simulink model "WBR_control"  (R2021b)
settings: Solver=ode4  StartTime=0.0  StopTime=12  FixedStep=1e-4  RelTol=1e-3
undefined symbols (not defined in the file): leg_controller, leg_l1, leg_l2, leg_model, leg_r1, leg_r2, locomotion_controller, param, sigbuilder_block, wheel_l, wheel_r, X, Y, Z
libraries: sm_lib x110, nesl_utility x29, slpidlib x2
(part 4 of 4)

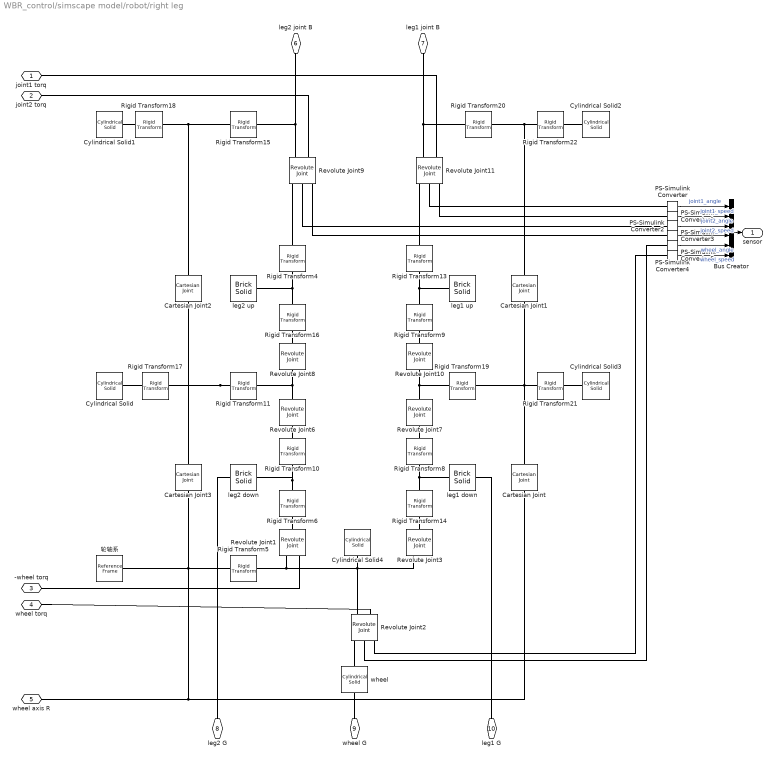
== system WBR_control/simscape model/robot/right leg ==
  Bus Creator : BusCreator  Inputs=6
  Cartesian Joint{,1..3} (4 alike) : sm_lib/Joints/Cartesian Joint  JointMode=Normal  SenseConstraintForce=off  SenseConstraintForceX=off  SenseConstraintForceY=off  SenseConstraintForceZ=off  SenseConstraintTorque=off  SenseConstraintTorqueX=off  SenseConstraintTorqueY=off  SenseConstraintTorqueZ=off  SenseTotalForce=off  SenseTotalForceX=off  SenseTotalForceY=off  SenseTotalForceZ=off  SenseTotalTorque=off  SenseTotalTorqueX=off  SenseTotalTorqueY=off  SenseTotalTorqueZ=off  CompositeWrenchDir=FollowerOnBase  CompositeWrenchFrame=BaseFrame  PxEquilibriumPosition=0  PxEquilibriumPositionUnits=m  PxSpringStiffness=0  PxSpringStiffnessUnits=N/m  PxDampingCoefficient=0  PxDampingCoefficientUnits=N/(m/s)  PxTorqueActuationMode=NoTorque  PxMotionActuationMode=ComputedMotion  PxSensePosition=off  PxSenseVelocity=off  PxSenseAcceleration=off  PxSenseTorqueForce=off  PxSenseLowerLimitTorqueForce=off  PxSenseUpperLimitTorqueForce=off  PxLowerLimitSpecify=off  PxLowerLimitBound=-1  PxLowerLimitBoundUnits=m  PxLowerLimitStiffness=1e6  PxLowerLimitStiffnessUnits=N/m  PxLowerLimitDamping=1e3  PxLowerLimitDampingUnits=N/(m/s)  PxLowerLimitTransitionRegionWidth=1e-4  PxLowerLimitTransitionRegionWidthUnits=m  PxUpperLimitSpecify=off  PxUpperLimitBound=1  PxUpperLimitBoundUnits=m  PxUpperLimitStiffness=1e6  PxUpperLimitStiffnessUnits=N/m  PxUpperLimitDamping=1e3  PxUpperLimitDampingUnits=N/(m/s)  PxUpperLimitTransitionRegionWidth=1e-4  PxUpperLimitTransitionRegionWidthUnits=m  PxPositionTargetSpecify=off  PxPositionTargetPriority=High  PxPositionTargetValue=0  PxPositionTargetValueUnits=m  PxVelocityTargetSpecify=off  PxVelocityTargetPriority=High  PxVelocityTargetValue=0  PxVelocityTargetValueUnits=m/s  PyEquilibriumPosition=0  PyEquilibriumPositionUnits=m  PySpringStiffness=0  PySpringStiffnessUnits=N/m  PyDampingCoefficient=0  PyDampingCoefficientUnits=N/(m/s)  PyTorqueActuationMode=NoTorque  PyMotionActuationMode=ComputedMotion  PySensePosition=off  PySenseVelocity=off  PySenseAcceleration=off  PySenseTorqueForce=off  PySenseLowerLimitTorqueForce=off  PySenseUpperLimitTorqueForce=off  PyLowerLimitSpecify=off  PyLowerLimitBound=-1  PyLowerLimitBoundUnits=m  PyLowerLimitStiffness=1e6  PyLowerLimitStiffnessUnits=N/m  PyLowerLimitDamping=1e3  PyLowerLimitDampingUnits=N/(m/s)  PyLowerLimitTransitionRegionWidth=1e-4  PyLowerLimitTransitionRegionWidthUnits=m  PyUpperLimitSpecify=off  PyUpperLimitBound=1  PyUpperLimitBoundUnits=m  PyUpperLimitStiffness=1e6  PyUpperLimitStiffnessUnits=N/m  PyUpperLimitDamping=1e3  PyUpperLimitDampingUnits=N/(m/s)  PyUpperLimitTransitionRegionWidth=1e-4  PyUpperLimitTransitionRegionWidthUnits=m  PyPositionTargetSpecify=off  PyPositionTargetPriority=High  PyPositionTargetValue=0  PyPositionTargetValueUnits=m  PyVelocityTargetSpecify=off  PyVelocityTargetPriority=High  PyVelocityTargetValue=0  PyVelocityTargetValueUnits=m/s  PzEquilibriumPosition=0  PzEquilibriumPositionUnits=m  PzSpringStiffness=0  PzSpringStiffnessUnits=N/m  PzDampingCoefficient=0  PzDampingCoefficientUnits=N/(m/s)  PzTorqueActuationMode=NoTorque  PzMotionActuationMode=ComputedMotion  PzSensePosition=off  PzSenseVelocity=off  PzSenseAcceleration=off  PzSenseTorqueForce=off  PzSenseLowerLimitTorqueForce=off  PzSenseUpperLimitTorqueForce=off  PzLowerLimitSpecify=off  PzLowerLimitBound=-1  PzLowerLimitBoundUnits=m  PzLowerLimitStiffness=1e6  PzLowerLimitStiffnessUnits=N/m  PzLowerLimitDamping=1e3  PzLowerLimitDampingUnits=N/(m/s)  PzLowerLimitTransitionRegionWidth=1e-4  PzLowerLimitTransitionRegionWidthUnits=m  PzUpperLimitSpecify=off  PzUpperLimitBound=1  PzUpperLimitBoundUnits=m  PzUpperLimitStiffness=1e6  PzUpperLimitStiffnessUnits=N/m  PzUpperLimitDamping=1e3  PzUpperLimitDampingUnits=N/(m/s)  PzUpperLimitTransitionRegionWidth=1e-4  PzUpperLimitTransitionRegionWidthUnits=m  PzPositionTargetSpecify=off  PzPositionTargetPriority=High  PzPositionTargetValue=0  PzPositionTargetValueUnits=m  PzVelocityTargetSpecify=off  PzVelocityTargetPriority=High  PzVelocityTargetValue=0  PzVelocityTargetValueUnits=m/s
  Cylindrical Solid{,1..3} (4 alike) : sm_lib/Body Elements/Cylindrical Solid  GraphicAmbientColor=[0.15 0.15 0.15 1.0]  BasedOnType=Mass  CenterOfMass=[0 0 0]  CenterOfMassUnits=m  GraphicDiffuseColor=[0.5 0.5 0.5]  CylinderLength=0.04  CylinderLengthUnits=m  CylinderRadius=0.025  CylinderRadiusUnits=m  Density=1e-5  DensityUnits=kg/m^3  DoExposeReferenceFrame=on  GraphicEmissiveColor=[0.0 0.0 0.0 1.0]  ExportEntireGeometry=off  SerializedFrames=<Frames/>  MarkerShape=Sphere  MarkerSize=10  GraphicType=FromGeometry  InertiaType=CalculateFromGeometry  Mass=1e-5  MassUnits=kg  MomentsOfInertia=[1 1 1]  MomentsOfInertiaUnits=kg*m^2  GraphicOpacity=1.0  ProductsOfInertia=[0 0 0]  ProductsOfInertiaUnits=kg*m^2  GraphicShininess=75  GraphicSpecularColor=[0.5 0.5 0.5 1.0]  GraphicVisPropType=SimpleVisualProperties
  Cylindrical Solid4 : sm_lib/Body Elements/Cylindrical Solid  GraphicAmbientColor=[0.15 0.15 0.15 1.0]  BasedOnType=Mass  CenterOfMass=[0 0 0]  CenterOfMassUnits=m  GraphicDiffuseColor=[0.5 0.5 0.5]  CylinderLength=0.04  CylinderLengthUnits=m  CylinderRadius=0.025  CylinderRadiusUnits=m  Density=1e-5  DensityUnits=kg/m^3  DoExposeReferenceFrame=on  GraphicEmissiveColor=[0.0 0.0 0.0 1.0]  ExportEntireGeometry=off  SerializedFrames=<Frames/>  MarkerShape=Sphere  MarkerSize=10  GraphicType=FromGeometry  InertiaType=Custom  Mass=0.9*2  MassUnits=kg  MomentsOfInertia=[1 1 1]*200e-6  MomentsOfInertiaUnits=kg*m^2  GraphicOpacity=1.0  ProductsOfInertia=[0 0 0]  ProductsOfInertiaUnits=kg*m^2  GraphicShininess=75  GraphicSpecularColor=[0.5 0.5 0.5 1.0]  GraphicVisPropType=SimpleVisualProperties
  PS-Simulink Converter{,1..5} (6 alike) : nesl_utility/PS-Simulink Converter  PhysicalDomain=network_engine_domain  SubClassName=ps_output  LeftPortType=input  RightPortType=output  PseudoPeriodic=off  Frequencies=[]  Unit=inherit  AffineConversion=off
      settings: SourceProductBaseCode=PW,SS
  Revolute Joint1 : sm_lib/Joints/Revolute Joint  JointMode=Normal  SenseConstraintForce=off  SenseConstraintForceX=off  SenseConstraintForceY=off  SenseConstraintForceZ=off  SenseConstraintTorque=off  SenseConstraintTorqueX=off  SenseConstraintTorqueY=off  SenseConstraintTorqueZ=off  SenseTotalForce=off  SenseTotalForceX=off  SenseTotalForceY=off  SenseTotalForceZ=off  SenseTotalTorque=off  SenseTotalTorqueX=off  SenseTotalTorqueY=off  SenseTotalTorqueZ=off  CompositeWrenchDir=FollowerOnBase  CompositeWrenchFrame=BaseFrame  EquilibriumPosition=0  EquilibriumPositionUnits=deg  SpringStiffness=0  SpringStiffnessUnits=N*m/deg  DampingCoefficient=0  DampingCoefficientUnits=N*m/(deg/s)  TorqueActuationMode=InputTorque  MotionActuationMode=ComputedMotion  SensePosition=off  SenseVelocity=off  SenseAcceleration=off  SenseTorqueForce=off  SenseLowerLimitTorqueForce=off  SenseUpperLimitTorqueForce=off  LowerLimitSpecify=off  LowerLimitBound=0  LowerLimitBoundUnits=deg  LowerLimitStiffness=1e4  LowerLimitStiffnessUnits=N*m/deg  LowerLimitDamping=10  LowerLimitDampingUnits=N*m/(deg/s)  LowerLimitTransitionRegionWidth=0.1  LowerLimitTransitionRegionWidthUnits=deg  UpperLimitSpecify=off  UpperLimitBound=120  UpperLimitBoundUnits=deg  UpperLimitStiffness=1e4  UpperLimitStiffnessUnits=N*m/deg  UpperLimitDamping=10  UpperLimitDampingUnits=N*m/(deg/s)  UpperLimitTransitionRegionWidth=0.1  UpperLimitTransitionRegionWidthUnits=deg  PositionTargetSpecify=on  PositionTargetPriority=Low  PositionTargetValue=45  PositionTargetValueUnits=deg  VelocityTargetSpecify=off  VelocityTargetPriority=High  VelocityTargetValue=0  VelocityTargetValueUnits=deg/s
  Revolute Joint10 : sm_lib/Joints/Revolute Joint  JointMode=Normal  SenseConstraintForce=off  SenseConstraintForceX=off  SenseConstraintForceY=off  SenseConstraintForceZ=off  SenseConstraintTorque=off  SenseConstraintTorqueX=off  SenseConstraintTorqueY=off  SenseConstraintTorqueZ=off  SenseTotalForce=off  SenseTotalForceX=off  SenseTotalForceY=off  SenseTotalForceZ=off  SenseTotalTorque=off  SenseTotalTorqueX=off  SenseTotalTorqueY=off  SenseTotalTorqueZ=off  CompositeWrenchDir=FollowerOnBase  CompositeWrenchFrame=BaseFrame  EquilibriumPosition=0  EquilibriumPositionUnits=deg  SpringStiffness=0  SpringStiffnessUnits=N*m/deg  DampingCoefficient=0  DampingCoefficientUnits=N*m/(deg/s)  TorqueActuationMode=NoTorque  MotionActuationMode=ComputedMotion  SensePosition=off  SenseVelocity=off  SenseAcceleration=off  SenseTorqueForce=off  SenseLowerLimitTorqueForce=off  SenseUpperLimitTorqueForce=off  LowerLimitSpecify=off  LowerLimitBound=60  LowerLimitBoundUnits=deg  LowerLimitStiffness=1e4  LowerLimitStiffnessUnits=N*m/deg  LowerLimitDamping=10  LowerLimitDampingUnits=N*m/(deg/s)  LowerLimitTransitionRegionWidth=0.1  LowerLimitTransitionRegionWidthUnits=deg  UpperLimitSpecify=off  UpperLimitBound=180  UpperLimitBoundUnits=deg  UpperLimitStiffness=1e4  UpperLimitStiffnessUnits=N*m/deg  UpperLimitDamping=10  UpperLimitDampingUnits=N*m/(deg/s)  UpperLimitTransitionRegionWidth=0.1  UpperLimitTransitionRegionWidthUnits=deg  PositionTargetSpecify=off  PositionTargetPriority=High  PositionTargetValue=180  PositionTargetValueUnits=deg  VelocityTargetSpecify=off  VelocityTargetPriority=High  VelocityTargetValue=0  VelocityTargetValueUnits=deg/s
  Revolute Joint11 : sm_lib/Joints/Revolute Joint  JointMode=Normal  SenseConstraintForce=off  SenseConstraintForceX=off  SenseConstraintForceY=off  SenseConstraintForceZ=off  SenseConstraintTorque=off  SenseConstraintTorqueX=off  SenseConstraintTorqueY=off  SenseConstraintTorqueZ=off  SenseTotalForce=off  SenseTotalForceX=off  SenseTotalForceY=off  SenseTotalForceZ=off  SenseTotalTorque=off  SenseTotalTorqueX=off  SenseTotalTorqueY=off  SenseTotalTorqueZ=off  CompositeWrenchDir=FollowerOnBase  CompositeWrenchFrame=BaseFrame  EquilibriumPosition=0  EquilibriumPositionUnits=deg  SpringStiffness=0  SpringStiffnessUnits=N*m/deg  DampingCoefficient=0  DampingCoefficientUnits=N*m/(deg/s)  TorqueActuationMode=InputTorque  MotionActuationMode=ComputedMotion  SensePosition=on  SenseVelocity=on  SenseAcceleration=off  SenseTorqueForce=off  SenseLowerLimitTorqueForce=off  SenseUpperLimitTorqueForce=off  LowerLimitSpecify=off  LowerLimitBound=60  LowerLimitBoundUnits=deg  LowerLimitStiffness=1e4  LowerLimitStiffnessUnits=N*m/deg  LowerLimitDamping=10  LowerLimitDampingUnits=N*m/(deg/s)  LowerLimitTransitionRegionWidth=0.1  LowerLimitTransitionRegionWidthUnits=deg  UpperLimitSpecify=off  UpperLimitBound=180  UpperLimitBoundUnits=deg  UpperLimitStiffness=1e4  UpperLimitStiffnessUnits=N*m/deg  UpperLimitDamping=10  UpperLimitDampingUnits=N*m/(deg/s)  UpperLimitTransitionRegionWidth=0.1  UpperLimitTransitionRegionWidthUnits=deg  PositionTargetSpecify=on  PositionTargetPriority=Low  PositionTargetValue=-20  PositionTargetValueUnits=deg  VelocityTargetSpecify=off  VelocityTargetPriority=High  VelocityTargetValue=0  VelocityTargetValueUnits=deg/s
  Revolute Joint2 : sm_lib/Joints/Revolute Joint  JointMode=Normal  SenseConstraintForce=off  SenseConstraintForceX=off  SenseConstraintForceY=off  SenseConstraintForceZ=off  SenseConstraintTorque=off  SenseConstraintTorqueX=off  SenseConstraintTorqueY=off  SenseConstraintTorqueZ=off  SenseTotalForce=off  SenseTotalForceX=off  SenseTotalForceY=off  SenseTotalForceZ=off  SenseTotalTorque=off  SenseTotalTorqueX=off  SenseTotalTorqueY=off  SenseTotalTorqueZ=off  CompositeWrenchDir=FollowerOnBase  CompositeWrenchFrame=BaseFrame  EquilibriumPosition=0  EquilibriumPositionUnits=deg  SpringStiffness=0  SpringStiffnessUnits=N*m/deg  DampingCoefficient=0  DampingCoefficientUnits=N*m/(deg/s)  TorqueActuationMode=InputTorque  MotionActuationMode=ComputedMotion  SensePosition=on  SenseVelocity=on  SenseAcceleration=off  SenseTorqueForce=off  SenseLowerLimitTorqueForce=off  SenseUpperLimitTorqueForce=off  LowerLimitSpecify=off  LowerLimitBound=-90  LowerLimitBoundUnits=deg  LowerLimitStiffness=1e4  LowerLimitStiffnessUnits=N*m/deg  LowerLimitDamping=10  LowerLimitDampingUnits=N*m/(deg/s)  LowerLimitTransitionRegionWidth=0.1  LowerLimitTransitionRegionWidthUnits=deg  UpperLimitSpecify=off  UpperLimitBound=90  UpperLimitBoundUnits=deg  UpperLimitStiffness=1e4  UpperLimitStiffnessUnits=N*m/deg  UpperLimitDamping=10  UpperLimitDampingUnits=N*m/(deg/s)  UpperLimitTransitionRegionWidth=0.1  UpperLimitTransitionRegionWidthUnits=deg  PositionTargetSpecify=off  PositionTargetPriority=High  PositionTargetValue=0  PositionTargetValueUnits=deg  VelocityTargetSpecify=off  VelocityTargetPriority=High  VelocityTargetValue=0  VelocityTargetValueUnits=deg/s
  Revolute Joint3 : sm_lib/Joints/Revolute Joint  JointMode=Normal  SenseConstraintForce=off  SenseConstraintForceX=off  SenseConstraintForceY=off  SenseConstraintForceZ=off  SenseConstraintTorque=off  SenseConstraintTorqueX=off  SenseConstraintTorqueY=off  SenseConstraintTorqueZ=off  SenseTotalForce=off  SenseTotalForceX=off  SenseTotalForceY=off  SenseTotalForceZ=off  SenseTotalTorque=off  SenseTotalTorqueX=off  SenseTotalTorqueY=off  SenseTotalTorqueZ=off  CompositeWrenchDir=FollowerOnBase  CompositeWrenchFrame=BaseFrame  EquilibriumPosition=0  EquilibriumPositionUnits=deg  SpringStiffness=0  SpringStiffnessUnits=N*m/deg  DampingCoefficient=0  DampingCoefficientUnits=N*m/(deg/s)  TorqueActuationMode=InputTorque  MotionActuationMode=ComputedMotion  SensePosition=off  SenseVelocity=off  SenseAcceleration=off  SenseTorqueForce=off  SenseLowerLimitTorqueForce=off  SenseUpperLimitTorqueForce=off  LowerLimitSpecify=off  LowerLimitBound=0  LowerLimitBoundUnits=deg  LowerLimitStiffness=1e4  LowerLimitStiffnessUnits=N*m/deg  LowerLimitDamping=10  LowerLimitDampingUnits=N*m/(deg/s)  LowerLimitTransitionRegionWidth=0.1  LowerLimitTransitionRegionWidthUnits=deg  UpperLimitSpecify=off  UpperLimitBound=120  UpperLimitBoundUnits=deg  UpperLimitStiffness=1e4  UpperLimitStiffnessUnits=N*m/deg  UpperLimitDamping=10  UpperLimitDampingUnits=N*m/(deg/s)  UpperLimitTransitionRegionWidth=0.1  UpperLimitTransitionRegionWidthUnits=deg  PositionTargetSpecify=on  PositionTargetPriority=Low  PositionTargetValue=135  PositionTargetValueUnits=deg  VelocityTargetSpecify=off  VelocityTargetPriority=High  VelocityTargetValue=0  VelocityTargetValueUnits=deg/s
  Revolute Joint6 : sm_lib/Joints/Revolute Joint  JointMode=Normal  SenseConstraintForce=off  SenseConstraintForceX=off  SenseConstraintForceY=off  SenseConstraintForceZ=off  SenseConstraintTorque=off  SenseConstraintTorqueX=off  SenseConstraintTorqueY=off  SenseConstraintTorqueZ=off  SenseTotalForce=off  SenseTotalForceX=off  SenseTotalForceY=off  SenseTotalForceZ=off  SenseTotalTorque=off  SenseTotalTorqueX=off  SenseTotalTorqueY=off  SenseTotalTorqueZ=off  CompositeWrenchDir=FollowerOnBase  CompositeWrenchFrame=BaseFrame  EquilibriumPosition=0  EquilibriumPositionUnits=deg  SpringStiffness=0  SpringStiffnessUnits=N*m/deg  DampingCoefficient=0  DampingCoefficientUnits=N*m/(deg/s)  TorqueActuationMode=NoTorque  MotionActuationMode=ComputedMotion  SensePosition=off  SenseVelocity=off  SenseAcceleration=off  SenseTorqueForce=off  SenseLowerLimitTorqueForce=off  SenseUpperLimitTorqueForce=off  LowerLimitSpecify=off  LowerLimitBound=60  LowerLimitBoundUnits=deg  LowerLimitStiffness=1e4  LowerLimitStiffnessUnits=N*m/deg  LowerLimitDamping=10  LowerLimitDampingUnits=N*m/(deg/s)  LowerLimitTransitionRegionWidth=0.1  LowerLimitTransitionRegionWidthUnits=deg  UpperLimitSpecify=off  UpperLimitBound=180  UpperLimitBoundUnits=deg  UpperLimitStiffness=1e4  UpperLimitStiffnessUnits=N*m/deg  UpperLimitDamping=10  UpperLimitDampingUnits=N*m/(deg/s)  UpperLimitTransitionRegionWidth=0.1  UpperLimitTransitionRegionWidthUnits=deg  PositionTargetSpecify=off  PositionTargetPriority=High  PositionTargetValue=0  PositionTargetValueUnits=deg  VelocityTargetSpecify=off  VelocityTargetPriority=High  VelocityTargetValue=0  VelocityTargetValueUnits=deg/s
  Revolute Joint7 : sm_lib/Joints/Revolute Joint  JointMode=Normal  SenseConstraintForce=off  SenseConstraintForceX=off  SenseConstraintForceY=off  SenseConstraintForceZ=off  SenseConstraintTorque=off  SenseConstraintTorqueX=off  SenseConstraintTorqueY=off  SenseConstraintTorqueZ=off  SenseTotalForce=off  SenseTotalForceX=off  SenseTotalForceY=off  SenseTotalForceZ=off  SenseTotalTorque=off  SenseTotalTorqueX=off  SenseTotalTorqueY=off  SenseTotalTorqueZ=off  CompositeWrenchDir=FollowerOnBase  CompositeWrenchFrame=BaseFrame  EquilibriumPosition=0  EquilibriumPositionUnits=deg  SpringStiffness=0  SpringStiffnessUnits=N*m/deg  DampingCoefficient=0  DampingCoefficientUnits=N*m/(deg/s)  TorqueActuationMode=NoTorque  MotionActuationMode=ComputedMotion  SensePosition=off  SenseVelocity=off  SenseAcceleration=off  SenseTorqueForce=off  SenseLowerLimitTorqueForce=off  SenseUpperLimitTorqueForce=off  LowerLimitSpecify=off  LowerLimitBound=60  LowerLimitBoundUnits=deg  LowerLimitStiffness=1e4  LowerLimitStiffnessUnits=N*m/deg  LowerLimitDamping=10  LowerLimitDampingUnits=N*m/(deg/s)  LowerLimitTransitionRegionWidth=0.1  LowerLimitTransitionRegionWidthUnits=deg  UpperLimitSpecify=off  UpperLimitBound=180  UpperLimitBoundUnits=deg  UpperLimitStiffness=1e4  UpperLimitStiffnessUnits=N*m/deg  UpperLimitDamping=10  UpperLimitDampingUnits=N*m/(deg/s)  UpperLimitTransitionRegionWidth=0.1  UpperLimitTransitionRegionWidthUnits=deg  PositionTargetSpecify=off  PositionTargetPriority=High  PositionTargetValue=0  PositionTargetValueUnits=deg  VelocityTargetSpecify=off  VelocityTargetPriority=High  VelocityTargetValue=0  VelocityTargetValueUnits=deg/s
  Revolute Joint8 : sm_lib/Joints/Revolute Joint  JointMode=Normal  SenseConstraintForce=off  SenseConstraintForceX=off  SenseConstraintForceY=off  SenseConstraintForceZ=off  SenseConstraintTorque=off  SenseConstraintTorqueX=off  SenseConstraintTorqueY=off  SenseConstraintTorqueZ=off  SenseTotalForce=off  SenseTotalForceX=off  SenseTotalForceY=off  SenseTotalForceZ=off  SenseTotalTorque=off  SenseTotalTorqueX=off  SenseTotalTorqueY=off  SenseTotalTorqueZ=off  CompositeWrenchDir=FollowerOnBase  CompositeWrenchFrame=BaseFrame  EquilibriumPosition=0  EquilibriumPositionUnits=deg  SpringStiffness=0  SpringStiffnessUnits=N*m/deg  DampingCoefficient=0  DampingCoefficientUnits=N*m/(deg/s)  TorqueActuationMode=NoTorque  MotionActuationMode=ComputedMotion  SensePosition=off  SenseVelocity=off  SenseAcceleration=off  SenseTorqueForce=off  SenseLowerLimitTorqueForce=off  SenseUpperLimitTorqueForce=off  LowerLimitSpecify=off  LowerLimitBound=60  LowerLimitBoundUnits=deg  LowerLimitStiffness=1e4  LowerLimitStiffnessUnits=N*m/deg  LowerLimitDamping=10  LowerLimitDampingUnits=N*m/(deg/s)  LowerLimitTransitionRegionWidth=0.1  LowerLimitTransitionRegionWidthUnits=deg  UpperLimitSpecify=off  UpperLimitBound=180  UpperLimitBoundUnits=deg  UpperLimitStiffness=1e4  UpperLimitStiffnessUnits=N*m/deg  UpperLimitDamping=10  UpperLimitDampingUnits=N*m/(deg/s)  UpperLimitTransitionRegionWidth=0.1  UpperLimitTransitionRegionWidthUnits=deg  PositionTargetSpecify=off  PositionTargetPriority=High  PositionTargetValue=180  PositionTargetValueUnits=deg  VelocityTargetSpecify=off  VelocityTargetPriority=High  VelocityTargetValue=0  VelocityTargetValueUnits=deg/s
  Revolute Joint9 : sm_lib/Joints/Revolute Joint  JointMode=Normal  SenseConstraintForce=off  SenseConstraintForceX=off  SenseConstraintForceY=off  SenseConstraintForceZ=off  SenseConstraintTorque=off  SenseConstraintTorqueX=off  SenseConstraintTorqueY=off  SenseConstraintTorqueZ=off  SenseTotalForce=off  SenseTotalForceX=off  SenseTotalForceY=off  SenseTotalForceZ=off  SenseTotalTorque=off  SenseTotalTorqueX=off  SenseTotalTorqueY=off  SenseTotalTorqueZ=off  CompositeWrenchDir=FollowerOnBase  CompositeWrenchFrame=BaseFrame  EquilibriumPosition=0  EquilibriumPositionUnits=deg  SpringStiffness=0  SpringStiffnessUnits=N*m/deg  DampingCoefficient=0  DampingCoefficientUnits=N*m/(deg/s)  TorqueActuationMode=InputTorque  MotionActuationMode=ComputedMotion  SensePosition=on  SenseVelocity=on  SenseAcceleration=off  SenseTorqueForce=off  SenseLowerLimitTorqueForce=off  SenseUpperLimitTorqueForce=off  LowerLimitSpecify=off  LowerLimitBound=60  LowerLimitBoundUnits=deg  LowerLimitStiffness=1e4  LowerLimitStiffnessUnits=N*m/deg  LowerLimitDamping=10  LowerLimitDampingUnits=N*m/(deg/s)  LowerLimitTransitionRegionWidth=0.1  LowerLimitTransitionRegionWidthUnits=deg  UpperLimitSpecify=off  UpperLimitBound=180  UpperLimitBoundUnits=deg  UpperLimitStiffness=1e4  UpperLimitStiffnessUnits=N*m/deg  UpperLimitDamping=10  UpperLimitDampingUnits=N*m/(deg/s)  UpperLimitTransitionRegionWidth=0.1  UpperLimitTransitionRegionWidthUnits=deg  PositionTargetSpecify=on  PositionTargetPriority=Low  PositionTargetValue=200  PositionTargetValueUnits=deg  VelocityTargetSpecify=off  VelocityTargetPriority=High  VelocityTargetValue=0  VelocityTargetValueUnits=deg/s
  Rigid Transform10 : sm_lib/Frames and Transforms/Rigid Transform  TranslationMethod=Cartesian  TranslationStandardOffset=0  TranslationLengthUnit=m  TranslationStandardAxis=+Z  TranslationCartesianOffset=[param.l_2d/2 0 0]  TranslationROffset=0  TranslationROffsetUnits=m  TranslationZOffset=0  TranslationZOffsetUnits=m  TranslationThetaOffset=0  TranslationThetaOffsetUnits=deg  RotationMethod=None  RotationAngleUnits=deg  RotationStandardAxis=+X  RotationAngle=90  RotationArbitraryAxis=[0 0 1]  FollAlignAxisA=+X  BaseAlignAxisA=+Y  FollAlignAxisB=+Y  BaseAlignAxisB=+Z  RotationSequenceAxes=FollowerAxes  RotationSequence=ZYX  RotationSequenceAngles=[135 0 0]  RotationSequenceAnglesUnits=deg  RotationMatrix=[-1 0 0; 0 0 1; 0 1 0]
  Rigid Transform{5,11,15,17..22} (9 alike) : sm_lib/Frames and Transforms/Rigid Transform  TranslationMethod=None  TranslationStandardOffset=0  TranslationLengthUnit=m  TranslationStandardAxis=+Z  TranslationCartesianOffset=[0 0 0]  TranslationROffset=0  TranslationROffsetUnits=m  TranslationZOffset=0  TranslationZOffsetUnits=m  TranslationThetaOffset=0  TranslationThetaOffsetUnits=deg  RotationMethod=RotationMatrix  RotationAngleUnits=deg  RotationStandardAxis=+X  RotationAngle=90  RotationArbitraryAxis=[0 0 1]  FollAlignAxisA=+X  BaseAlignAxisA=+Y  FollAlignAxisB=+Y  BaseAlignAxisB=+Z  RotationSequenceAxes=FollowerAxes  RotationSequence=XYX  RotationSequenceAngles=[0 0 0]  RotationSequenceAnglesUnits=deg  RotationMatrix=[-1 0 0; 0 0 1; 0 1 0]
  Rigid Transform13 : sm_lib/Frames and Transforms/Rigid Transform  TranslationMethod=Cartesian  TranslationStandardOffset=0  TranslationLengthUnit=m  TranslationStandardAxis=+Z  TranslationCartesianOffset=[param.l_1u/2 0 0]  TranslationROffset=0  TranslationROffsetUnits=m  TranslationZOffset=0  TranslationZOffsetUnits=m  TranslationThetaOffset=0  TranslationThetaOffsetUnits=deg  RotationMethod=None  RotationAngleUnits=deg  RotationStandardAxis=+X  RotationAngle=90  RotationArbitraryAxis=[0 0 1]  FollAlignAxisA=+X  BaseAlignAxisA=+Y  FollAlignAxisB=+Y  BaseAlignAxisB=+Z  RotationSequenceAxes=FollowerAxes  RotationSequence=ZYX  RotationSequenceAngles=[135 0 0]  RotationSequenceAnglesUnits=deg  RotationMatrix=[-1 0 0; 0 0 1; 0 1 0]
  Rigid Transform14 : sm_lib/Frames and Transforms/Rigid Transform  TranslationMethod=Cartesian  TranslationStandardOffset=0  TranslationLengthUnit=m  TranslationStandardAxis=+Z  TranslationCartesianOffset=[param.l_1d/2 0 0]  TranslationROffset=0  TranslationROffsetUnits=m  TranslationZOffset=0  TranslationZOffsetUnits=m  TranslationThetaOffset=0  TranslationThetaOffsetUnits=deg  RotationMethod=None  RotationAngleUnits=deg  RotationStandardAxis=+X  RotationAngle=90  RotationArbitraryAxis=[0 0 1]  FollAlignAxisA=+X  BaseAlignAxisA=+Y  FollAlignAxisB=+Y  BaseAlignAxisB=+Z  RotationSequenceAxes=FollowerAxes  RotationSequence=ZYX  RotationSequenceAngles=[135 0 0]  RotationSequenceAnglesUnits=deg  RotationMatrix=[-1 0 0; 0 0 1; 0 1 0]
  Rigid Transform16 : sm_lib/Frames and Transforms/Rigid Transform  TranslationMethod=Cartesian  TranslationStandardOffset=0  TranslationLengthUnit=m  TranslationStandardAxis=+Z  TranslationCartesianOffset=[param.l_2u/2 0 0]  TranslationROffset=0  TranslationROffsetUnits=m  TranslationZOffset=0  TranslationZOffsetUnits=m  TranslationThetaOffset=0  TranslationThetaOffsetUnits=deg  RotationMethod=None  RotationAngleUnits=deg  RotationStandardAxis=+X  RotationAngle=90  RotationArbitraryAxis=[0 0 1]  FollAlignAxisA=+X  BaseAlignAxisA=+Y  FollAlignAxisB=+Y  BaseAlignAxisB=+Z  RotationSequenceAxes=FollowerAxes  RotationSequence=ZYX  RotationSequenceAngles=[135 0 0]  RotationSequenceAnglesUnits=deg  RotationMatrix=[-1 0 0; 0 0 1; 0 1 0]
  Rigid Transform4 : sm_lib/Frames and Transforms/Rigid Transform  TranslationMethod=Cartesian  TranslationStandardOffset=0  TranslationLengthUnit=m  TranslationStandardAxis=+Z  TranslationCartesianOffset=[param.l_2u/2 0 0]  TranslationROffset=0  TranslationROffsetUnits=m  TranslationZOffset=0  TranslationZOffsetUnits=m  TranslationThetaOffset=0  TranslationThetaOffsetUnits=deg  RotationMethod=None  RotationAngleUnits=deg  RotationStandardAxis=+X  RotationAngle=90  RotationArbitraryAxis=[0 0 1]  FollAlignAxisA=+X  BaseAlignAxisA=+Y  FollAlignAxisB=+Y  BaseAlignAxisB=+Z  RotationSequenceAxes=FollowerAxes  RotationSequence=ZYX  RotationSequenceAngles=[135 0 0]  RotationSequenceAnglesUnits=deg  RotationMatrix=[-1 0 0; 0 0 1; 0 1 0]
  Rigid Transform6 : sm_lib/Frames and Transforms/Rigid Transform  TranslationMethod=Cartesian  TranslationStandardOffset=0  TranslationLengthUnit=m  TranslationStandardAxis=+Z  TranslationCartesianOffset=[param.l_2d/2 0 0]  TranslationROffset=0  TranslationROffsetUnits=m  TranslationZOffset=0  TranslationZOffsetUnits=m  TranslationThetaOffset=0  TranslationThetaOffsetUnits=deg  RotationMethod=None  RotationAngleUnits=deg  RotationStandardAxis=+X  RotationAngle=90  RotationArbitraryAxis=[0 0 1]  FollAlignAxisA=+X  BaseAlignAxisA=+Y  FollAlignAxisB=+Y  BaseAlignAxisB=+Z  RotationSequenceAxes=FollowerAxes  RotationSequence=ZYX  RotationSequenceAngles=[135 0 0]  RotationSequenceAnglesUnits=deg  RotationMatrix=[-1 0 0; 0 0 1; 0 1 0]
  Rigid Transform8 : sm_lib/Frames and Transforms/Rigid Transform  TranslationMethod=Cartesian  TranslationStandardOffset=0  TranslationLengthUnit=m  TranslationStandardAxis=+Z  TranslationCartesianOffset=[param.l_1d/2 0 0]  TranslationROffset=0  TranslationROffsetUnits=m  TranslationZOffset=0  TranslationZOffsetUnits=m  TranslationThetaOffset=0  TranslationThetaOffsetUnits=deg  RotationMethod=None  RotationAngleUnits=deg  RotationStandardAxis=+X  RotationAngle=90  RotationArbitraryAxis=[0 0 1]  FollAlignAxisA=+X  BaseAlignAxisA=+Y  FollAlignAxisB=+Y  BaseAlignAxisB=+Z  RotationSequenceAxes=FollowerAxes  RotationSequence=ZYX  RotationSequenceAngles=[135 0 0]  RotationSequenceAnglesUnits=deg  RotationMatrix=[-1 0 0; 0 0 1; 0 1 0]
  Rigid Transform9 : sm_lib/Frames and Transforms/Rigid Transform  TranslationMethod=Cartesian  TranslationStandardOffset=0  TranslationLengthUnit=m  TranslationStandardAxis=+Z  TranslationCartesianOffset=[param.l_1u/2 0 0]  TranslationROffset=0  TranslationROffsetUnits=m  TranslationZOffset=0  TranslationZOffsetUnits=m  TranslationThetaOffset=0  TranslationThetaOffsetUnits=deg  RotationMethod=None  RotationAngleUnits=deg  RotationStandardAxis=+X  RotationAngle=90  RotationArbitraryAxis=[0 0 1]  FollAlignAxisA=+X  BaseAlignAxisA=+Y  FollAlignAxisB=+Y  BaseAlignAxisB=+Z  RotationSequenceAxes=FollowerAxes  RotationSequence=ZYX  RotationSequenceAngles=[135 0 0]  RotationSequenceAnglesUnits=deg  RotationMatrix=[-1 0 0; 0 0 1; 0 1 0]
  leg1 down : sm_lib/Body Elements/Brick Solid  GraphicAmbientColor=[0.15 0.15 0.15 1.0]  BasedOnType=Mass  BrickDimensions=[param.l_1d 0.05 0.04]  BrickDimensionUnits=m  CenterOfMass=[0 0 0]  CenterOfMassUnits=m  GraphicDiffuseColor=[0.5 0.5 0.5]  Density=1000  DensityUnits=kg/m^3  DoExposeReferenceFrame=on  GraphicEmissiveColor=[0.0 0.0 0.0 1.0]  ExportEntireGeometry=on  SerializedFrames=<Frames/>  MarkerShape=Sphere  MarkerSize=10  GraphicType=FromGeometry  InertiaType=Custom  Mass=0.385  MassUnits=kg  MomentsOfInertia=[600 2200 3855]*1e-6  MomentsOfInertiaUnits=kg*m^2  GraphicOpacity=1.0  ProductsOfInertia=[0 0 0]  ProductsOfInertiaUnits=kg*m^2  GraphicShininess=75  GraphicSpecularColor=[0.5 0.5 0.5 1.0]  GraphicVisPropType=SimpleVisualProperties
  leg1 up : sm_lib/Body Elements/Brick Solid  GraphicAmbientColor=[0.15 0.15 0.15 1.0]  BasedOnType=Mass  BrickDimensions=[param.l_1u 0.05 0.04]  BrickDimensionUnits=m  CenterOfMass=[0 0 0]  CenterOfMassUnits=m  GraphicDiffuseColor=[0.5 0.5 0.5]  Density=1000  DensityUnits=kg/m^3  DoExposeReferenceFrame=on  GraphicEmissiveColor=[0.0 0.0 0.0 1.0]  ExportEntireGeometry=on  SerializedFrames=<Frames/>  MarkerShape=Sphere  MarkerSize=10  GraphicType=FromGeometry  InertiaType=Custom  Mass=0.385  MassUnits=kg  MomentsOfInertia=[400 1200 1680]*1e-6  MomentsOfInertiaUnits=kg*m^2  GraphicOpacity=1.0  ProductsOfInertia=[0 0 0]  ProductsOfInertiaUnits=kg*m^2  GraphicShininess=75  GraphicSpecularColor=[0.5 0.5 0.5 1.0]  GraphicVisPropType=SimpleVisualProperties
  leg2 down : sm_lib/Body Elements/Brick Solid  GraphicAmbientColor=[0.15 0.15 0.15 1.0]  BasedOnType=Mass  BrickDimensions=[param.l_2d 0.05 0.04]  BrickDimensionUnits=m  CenterOfMass=[0 0 0]  CenterOfMassUnits=m  GraphicDiffuseColor=[0.5 0.5 0.5]  Density=1000  DensityUnits=kg/m^3  DoExposeReferenceFrame=on  GraphicEmissiveColor=[0.0 0.0 0.0 1.0]  ExportEntireGeometry=on  SerializedFrames=<Frames/>  MarkerShape=Sphere  MarkerSize=10  GraphicType=FromGeometry  InertiaType=Custom  Mass=0.385  MassUnits=kg  MomentsOfInertia=[600 2200 3855]*1e-6  MomentsOfInertiaUnits=kg*m^2  GraphicOpacity=1.0  ProductsOfInertia=[0 0 0]  ProductsOfInertiaUnits=kg*m^2  GraphicShininess=75  GraphicSpecularColor=[0.5 0.5 0.5 1.0]  GraphicVisPropType=SimpleVisualProperties
  leg2 up : sm_lib/Body Elements/Brick Solid  GraphicAmbientColor=[0.15 0.15 0.15 1.0]  BasedOnType=Mass  BrickDimensions=[param.l_2u 0.05 0.04]  BrickDimensionUnits=m  CenterOfMass=[0 0 0]  CenterOfMassUnits=m  GraphicDiffuseColor=[0.5 0.5 0.5]  Density=1000  DensityUnits=kg/m^3  DoExposeReferenceFrame=on  GraphicEmissiveColor=[0.0 0.0 0.0 1.0]  ExportEntireGeometry=on  SerializedFrames=<Frames/>  MarkerShape=Sphere  MarkerSize=10  GraphicType=FromGeometry  InertiaType=Custom  Mass=0.385  MassUnits=kg  MomentsOfInertia=[400 1200 1680]*1e-6  MomentsOfInertiaUnits=kg*m^2  GraphicOpacity=1.0  ProductsOfInertia=[0 0 0]  ProductsOfInertiaUnits=kg*m^2  GraphicShininess=75  GraphicSpecularColor=[0.5 0.5 0.5 1.0]  GraphicVisPropType=SimpleVisualProperties
  wheel : sm_lib/Body Elements/Cylindrical Solid  GraphicAmbientColor=[0.15 0.15 0.15 1.0]  BasedOnType=Density  CenterOfMass=[0 0 0]  CenterOfMassUnits=m  GraphicDiffuseColor=[1.0 1.0 0.8]  CylinderLength=0.042  CylinderLengthUnits=m  CylinderRadius=param.R_w  CylinderRadiusUnits=m  Density=1000  DensityUnits=kg/m^3  DoExposeReferenceFrame=on  GraphicEmissiveColor=[0.0 0.0 0.0 1.0]  ExportEntireGeometry=on  SerializedFrames=<Frames/>  MarkerShape=Sphere  MarkerSize=10  GraphicType=FromGeometry  InertiaType=Custom  Mass=param.m_w  MassUnits=kg  MomentsOfInertia=[400e-6 400e-6 param.I_w]  MomentsOfInertiaUnits=kg*m^2  GraphicOpacity=1.0  ProductsOfInertia=[0 0 0]  ProductsOfInertiaUnits=kg*m^2  GraphicShininess=75  GraphicSpecularColor=[0.5 0.5 0.5 1.0]  GraphicVisPropType=SimpleVisualProperties
  轮轴系 : sm_lib/Frames and Transforms/Reference Frame
  joint1 torq : PMIOPort  Side=Left
  joint2 torq : PMIOPort  Port=2  Side=Left
  -wheel torq : PMIOPort  Port=3  Side=Left
  wheel torq : PMIOPort  Port=4  Side=Left
  wheel axis R : PMIOPort  Port=5  Side=Left
  leg2 joint B : PMIOPort  Port=6  Side=Left
  leg1 joint B : PMIOPort  Port=7  Side=Left
  leg2 G : PMIOPort  Port=8  Side=Right
  wheel G : PMIOPort  Port=9  Side=Right
  leg1 G : PMIOPort  Port=10  Side=Right
  sensor : Outport
  wires:
  PS-Simulink Converter3/1 -> Bus Creator/4  "joint2_speed"
  PS-Simulink Converter2/1 -> Bus Creator/3  "joint2_angle"
  PS-Simulink Converter1/1 -> Bus Creator/2  "joint1_speed"
  PS-Simulink Converter/1 -> Bus Creator/1  "joint1_angle"
  PS-Simulink Converter4/1 -> Bus Creator/5  "wheel_angle"
  PS-Simulink Converter5/1 -> Bus Creator/6  "wheel_speed"
  Bus Creator/1 -> sensor/1
  connections:
  Revolute Joint6/RConn1 -- Rigid Transform10/RConn1
  wheel/LConn1 -- wheel G/RConn1
  Revolute Joint3/LConn1 -- Revolute Joint2/LConn1 -- Revolute Joint1/LConn1 -- Rigid Transform5/RConn1 -- Cylindrical Solid4/RConn1
  Rigid Transform8/LConn1 -- leg1 down/RConn1 -- Rigid Transform14/RConn1
  Rigid Transform6/LConn1 -- Revolute Joint1/RConn1
  Revolute Joint6/LConn1 -- Revolute Joint8/LConn1 -- Rigid Transform11/RConn1
  Rigid Transform11/LConn1 -- Cartesian Joint3/RConn1 -- Rigid Transform17/LConn1 -- Cartesian Joint2/LConn1
  Rigid Transform20/LConn1 -- Rigid Transform22/LConn1 -- Cartesian Joint1/RConn1
  Cartesian Joint1/LConn1 -- Cartesian Joint/RConn1 -- Rigid Transform19/LConn1 -- Rigid Transform21/LConn1
  Revolute Joint10/LConn1 -- Revolute Joint7/LConn1 -- Rigid Transform19/RConn1
  Revolute Joint2/RConn1 -- wheel/RConn1
  Rigid Transform20/RConn1 -- leg1 joint B/RConn1 -- Revolute Joint11/LConn1
  wheel torq/RConn1 -- Revolute Joint2/LConn2
  Rigid Transform16/RConn1 -- leg2 up/RConn1 -- Rigid Transform4/LConn1
  Rigid Transform13/LConn1 -- leg1 up/RConn1 -- Rigid Transform9/RConn1
  Revolute Joint7/RConn1 -- Rigid Transform8/RConn1
  Rigid Transform6/RConn1 -- Rigid Transform10/LConn1 -- leg2 down/RConn1
  轮轴系/RConn1 -- Cartesian Joint3/LConn1 -- Rigid Transform5/LConn1 -- Cartesian Joint/LConn1 -- wheel axis R/RConn1
  Rigid Transform9/LConn1 -- Revolute Joint10/RConn1
  -wheel torq/RConn1 -- Revolute Joint1/LConn2
  Rigid Transform14/LConn1 -- Revolute Joint3/RConn1
  Rigid Transform4/RConn1 -- Revolute Joint9/RConn1
  Cylindrical Solid3/RConn1 -- Rigid Transform21/RConn1
  joint1 torq/RConn1 -- Revolute Joint11/LConn2
  Cylindrical Solid/RConn1 -- Rigid Transform17/RConn1
  Revolute Joint11/RConn1 -- Rigid Transform13/RConn1
  Rigid Transform16/LConn1 -- Revolute Joint8/RConn1
  Rigid Transform15/RConn1 -- leg2 joint B/RConn1 -- Revolute Joint9/LConn1
  leg2 down/LConn1 -- leg2 G/RConn1
  leg1 down/LConn1 -- leg1 G/RConn1
  Rigid Transform18/LConn1 -- Rigid Transform15/LConn1 -- Cartesian Joint2/RConn1
  Cylindrical Solid1/RConn1 -- Rigid Transform18/RConn1
  Rigid Transform22/RConn1 -- Cylindrical Solid2/RConn1
  joint2 torq/RConn1 -- Revolute Joint9/LConn2
  PS-Simulink Converter1/LConn1 -- Revolute Joint11/RConn3
  PS-Simulink Converter/LConn1 -- Revolute Joint11/RConn2
  PS-Simulink Converter2/LConn1 -- Revolute Joint9/RConn2
  PS-Simulink Converter3/LConn1 -- Revolute Joint9/RConn3
  PS-Simulink Converter5/LConn1 -- Revolute Joint2/RConn3
  PS-Simulink Converter4/LConn1 -- Revolute Joint2/RConn2

== matlab function WBR_control/observer/observer function ==
  data: theta_wl input; theta_wl_D1 input; theta_wr input; x output; psi output; theta_wr_D1 input; theta_b input; theta_b_D1 input; phi input; phi_D1 input; psi input; theta_bll input; theta_bll_D1 input; theta_blr input; theta_blr_D1 input; R_w input
function [x,psi] = sensor2state(theta_wl,theta_wl_D1, ...
                                theta_wr,theta_wr_D1, ...
                                theta_b,theta_b_D1, ...
                                phi,phi_D1, ...
                                psi, ...
                                theta_bll,theta_bll_D1, ...
                                theta_blr,theta_blr_D1, ...
                                R_w)
% sensor data to state

s = R_w/2*(theta_wl+theta_wr);
s_D1 = R_w/2*(theta_wl_D1+theta_wr_D1);
theta_ll = theta_b+theta_bll;
theta_ll_D1 = theta_b_D1+theta_bll_D1;
theta_lr = theta_b+theta_blr;
theta_lr_D1 = theta_b_D1+theta_blr_D1;
x = [s;s_D1;phi;phi_D1;theta_ll;theta_ll_D1;theta_lr;theta_lr_D1;theta_b;theta_b_D1];

== matlab function WBR_control/observer/left leg forward kinematic ==
  data: phi1 input; phi2 input; la input; lu input; l output; theta output; k_xe input; k_ye input; xe output; ye output; xi output; yi output
function [l,theta,xe,ye,xi,yi] = legFkine(phi1,phi2,la,lu,k_xe,k_ye)
% forward kinematic of leg
% note: l_1a=l_2a=la, l_1u=l_2u=lu, l_1d=l_2d=ld

xi = [la-lu*cos(phi1)
      la-lu*cos(phi2)];
yi = [lu*sin(phi1)
      lu*sin(phi2)];
xe = [1,phi1,phi2,phi1^2,phi2^2,phi1*phi2]*k_xe;
ye = [1,phi1,phi2,phi1^2,phi2^2,phi1*phi2]*k_ye;
l = sqrt(xe^2+ye^2);
theta = atan2(xe,ye);

== matlab function WBR_control/observer/right leg forward kinematic ==
  data: phi1 input; phi2 input; la input; lu input; l output; theta output; k_xe input; k_ye input; xe output; ye output; xi output; yi output
function [l,theta,xe,ye,xi,yi] = legFkine(phi1,phi2,la,lu,k_xe,k_ye)
% forward kinematic of leg
% note: l_1a=l_2a=la, l_1u=l_2u=lu, l_1d=l_2d=ld

xi = [la-lu*cos(phi1)
      la-lu*cos(phi2)];
yi = [lu*sin(phi1)
      lu*sin(phi2)];
xe = [1,phi1,phi2,phi1^2,phi2^2,phi1*phi2]*k_xe;
ye = [1,phi1,phi2,phi1^2,phi2^2,phi1*phi2]*k_ye;
l = sqrt(xe^2+ye^2);
theta = atan2(xe,ye);

== matlab function WBR_control/controller/leg_controller/gravity feedfoward force ==
  data: F output; m_b input; m_l input; eta_l input
function F = gravity_ff(m_b,m_l,eta_l)
% feedforward support force of leg against body gravity

F = (m_b/2+eta_l*m_l)*9.81;

== matlab function WBR_control/observer/right leg jacobian ==
  data: phi1 input; phi2 input; l input; J output; theta input; xe input; ye input; xi input; yi input; lu input
function J = legJacob(phi1,phi2,l,theta,xe,ye,xi,yi,lu)
% transpose of jacobian matrix of leg mechanism
% note: l_1a=l_2a=la, l_1u=l_2u=lu, l_1d=l_2d=ld

phi = [phi1;phi2];
Pphi1Pl = @(l,theta,phi,xe,ye,xi,yi,li_u)1/li_u(1) ...
                *((xe+xi(1))*sin(theta)+(ye-yi(1))*cos(theta)) ...
                /(-(xe+xi(1))*sin(phi(1))+(ye-yi(1))*cos(phi(1)));
Pphi1Ptheta = @(l,theta,phi,xe,ye,xi,yi,li_u)l/li_u(1) ...
                *((xe+xi(1))*cos(theta)-(ye-yi(1))*sin(theta)) ...
                /(-(xe+xi(1))*sin(phi(1))+(ye-yi(1))*cos(phi(1)));
Pphi2Pl = @(l,theta,phi,xe,ye,xi,yi,li_u)1/li_u(2) ...
                *((xe-xi(2))*sin(theta)+(ye-yi(2))*cos(theta)) ...
                /((xe-xi(2))*sin(phi(2))+(ye-yi(2))*cos(phi(2)));
Pphi2Ptheta = @(l,theta,phi,xe,ye,xi,yi,li_u)l/li_u(2) ...
                *((xe-xi(2))*cos(theta)-(ye-yi(2))*sin(theta)) ...
                /((xe-xi(2))*sin(phi(2))+(ye-yi(2))*cos(phi(2)));
J = inv([Pphi1Pl(l,theta,phi,xe,ye,xi,yi,[lu;lu]), ...
         Pphi1Ptheta(l,theta,phi,xe,ye,xi,yi,[lu;lu]); ...
         Pphi2Pl(l,theta,phi,xe,ye,xi,yi,[lu;lu]), ...
         Pphi2Ptheta(l,theta,phi,xe,ye,xi,yi,[lu;lu])]);

== matlab function WBR_control/observer/left leg jacobian ==
  data: phi1 input; phi2 input; l input; J output; theta input; xe input; ye input; xi input; yi input; lu input
function J = legJacob(phi1,phi2,l,theta,xe,ye,xi,yi,lu)
% transpose of jacobian matrix of leg mechanism
% note: l_1a=l_2a=la, l_1u=l_2u=lu, l_1d=l_2d=ld

phi = [phi1;phi2];
Pphi1Pl = @(l,theta,phi,xe,ye,xi,yi,li_u)1/li_u(1) ...
                *((xe+xi(1))*sin(theta)+(ye-yi(1))*cos(theta)) ...
                /(-(xe+xi(1))*sin(phi(1))+(ye-yi(1))*cos(phi(1)));
Pphi1Ptheta = @(l,theta,phi,xe,ye,xi,yi,li_u)l/li_u(1) ...
                *((xe+xi(1))*cos(theta)-(ye-yi(1))*sin(theta)) ...
                /(-(xe+xi(1))*sin(phi(1))+(ye-yi(1))*cos(phi(1)));
Pphi2Pl = @(l,theta,phi,xe,ye,xi,yi,li_u)1/li_u(2) ...
                *((xe-xi(2))*sin(theta)+(ye-yi(2))*cos(theta)) ...
                /((xe-xi(2))*sin(phi(2))+(ye-yi(2))*cos(phi(2)));
Pphi2Ptheta = @(l,theta,phi,xe,ye,xi,yi,li_u)l/li_u(2) ...
                *((xe-xi(2))*cos(theta)-(ye-yi(2))*sin(theta)) ...
                /((xe-xi(2))*sin(phi(2))+(ye-yi(2))*cos(phi(2)));
J = inv([Pphi1Pl(l,theta,phi,xe,ye,xi,yi,[lu;lu]), ...
         Pphi1Ptheta(l,theta,phi,xe,ye,xi,yi,[lu;lu]); ...
         Pphi2Pl(l,theta,phi,xe,ye,xi,yi,[lu;lu]), ...
         Pphi2Ptheta(l,theta,phi,xe,ye,xi,yi,[lu;lu])]);

== matlab function WBR_control/controller/locomotion_controller/leg length to K ==
  data: ll input; lr input; K output; KK input
function K = l2K(ll,lr,KK)

% K = KK(:,:,1)+KK(:,:,2)*ll+KK(:,:,3)*ll^2+KK(:,:,4)*lr+KK(:,:,5)*lr^2+KK(:,:,6)*ll*lr;
K = KK(:,:,1)+KK(:,:,2)*ll+KK(:,:,3)*lr;

== matlab function WBR_control/controller/leg_controller/inertia feedforward force ==
  data: x input; F output; l input; m_b input; m_l input; R_l input; eta_l input
function F = inertial_ff(x,l,m_b,m_l,R_l,eta_l)
% feedforward support force of leg against lateral moment of inertia

s_D1 = x(2);
phi_D1 = x(4);
F = (m_b/2+eta_l*m_l)*l/(2*R_l)*phi_D1*s_D1;
